simulink model "dc_voltage_control_A"  (R2018b)
settings: Solver=ode45  StartTime=0.0  StopTime=90  MaxStep=100e-6  RelTol=1e-3
PreLoadFcn:
  | load_system('../simulink_reference_models/test_sequence_lib');
InitFcn:
  | close all
  | clear all
  | 
  | T_CNTL = 1/5e3;
  | 
  | VLL_NOM = 480;
  | F_NOM = 60;
  | VLL_INV_NOM = VLL_NOM;
  | S_RATED = 1e6;
  | I_BASE = S_RATED / (sqrt(3) * VLL_NOM);
  | 
  | V_LVDC_NOM = 0.0; % to make cap voltage start from 0
  | C_DC = 50e-3;
libraries: simulink x12, test_sequence_lib x6, controls_element_lib x1
settings Model: SimulationMode=accelerator  Creator=HussamAlatrash  LastModifiedBy=ahhei
settings DataIOCC: ReturnWorkspaceOutputs=on
settings DebuggingCC: UnconnectedInputMsg=none  UnconnectedOutputMsg=none  UnconnectedLineMsg=none
settings ModelReferenceCC: EnableRefExpFcnMdlSchedulingChecks=off
settings RTWCC: Description=Generic Real-Time Target
settings ConfigComp: CovBoundaryAbsTol=1.0e-5

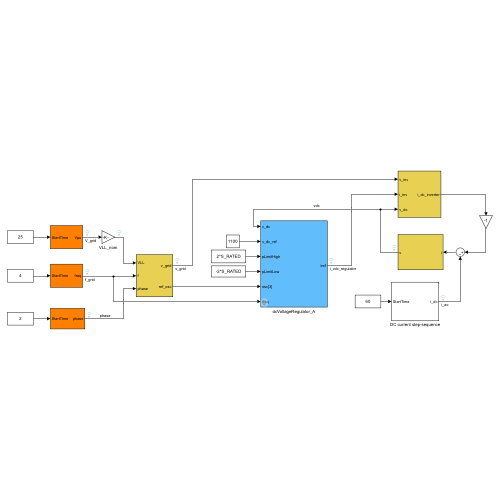
[thumbnail: Simulink's stored preview of the top-level diagram]
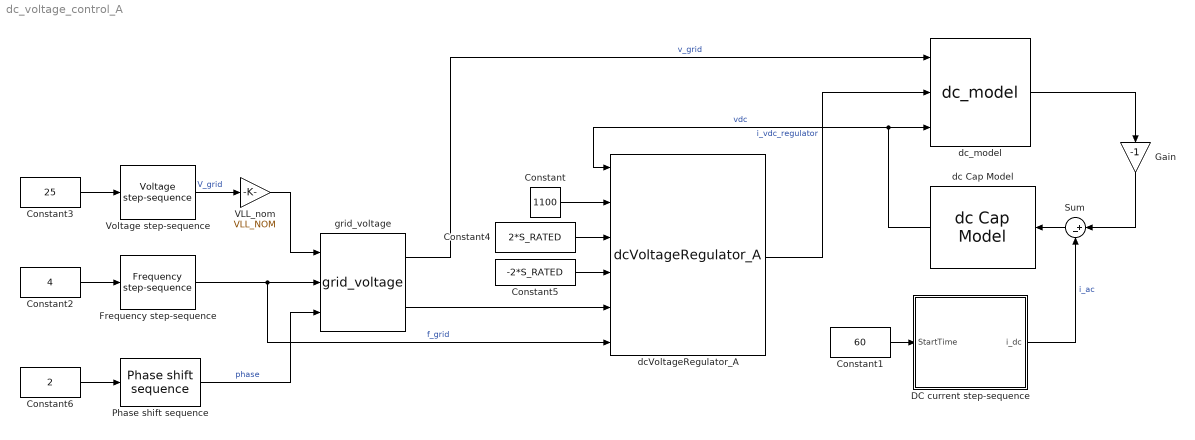
== system dc_voltage_control_A ==
  Constant : Constant  Value=1100
  Constant1 : Constant  Value=60
  Constant2 : Constant  Value=4
  Constant3 : Constant  Value=25
  Constant4 : Constant  Value=2*S_RATED
  Constant5 : Constant  Value=-2*S_RATED
  Constant6 : Constant  Value=2
  DC current step-sequence : Subsystem
  Frequency step-sequence : test_sequence_lib/Frequency step-sequence  SystemSampleTime=-1  EmptyChoice=off  PassThrough=off  PassThroughVariantControl=(default)  EmptyChoiceVariantControl=(default)  Latency=0  AutoFrameSizeCalculation=off
  Gain : Gain  Gain=-1
  Phase shift sequence : test_sequence_lib/Phase shift sequence  SystemSampleTime=-1  EmptyChoice=off  PassThrough=off  PassThroughVariantControl=(default)  EmptyChoiceVariantControl=(default)  Latency=0  AutoFrameSizeCalculation=off
  Sum : Sum  Inputs=|+-
  VLL_nom : Gain  Gain=VLL_NOM
  Voltage step-sequence : test_sequence_lib/Voltage step-sequence  SystemSampleTime=-1  EmptyChoice=off  PassThrough=off  PassThroughVariantControl=(default)  EmptyChoiceVariantControl=(default)  Latency=0  AutoFrameSizeCalculation=off
  dc Cap Model : test_sequence_lib/dc Cap Model  SystemSampleTime=-1  EmptyChoice=off  PassThrough=off  PassThroughVariantControl=(default)  EmptyChoiceVariantControl=(default)  Latency=0  AutoFrameSizeCalculation=off
  dcVoltageRegulator_A : controls_element_lib/dcVoltageRegulator_A  kp=20e3  kSlowPath=0  wSlowPath=5  pLimitExternalMinimum=0  vdc_deadband=0  VllRated=VLL_INV_NOM
  dc_model : test_sequence_lib/dc_model  SystemSampleTime=-1  EmptyChoice=off  PassThrough=off  PassThroughVariantControl=(default)  EmptyChoiceVariantControl=(default)  Latency=0  AutoFrameSizeCalculation=off
  grid_voltage : test_sequence_lib/grid_voltage  SystemSampleTime=-1  EmptyChoice=off  PassThrough=off  PassThroughVariantControl=(default)  EmptyChoiceVariantControl=(default)  Latency=0  AutoFrameSizeCalculation=off
  wires:
  Constant2/1 -> Frequency step-sequence/1
  Constant3/1 -> Voltage step-sequence/1
  Constant6/1 -> Phase shift sequence/1
  VLL_nom/1 -> grid_voltage/1
  Voltage step-sequence/1 -> VLL_nom/1  "V_grid"
  Frequency step-sequence/1 -> dcVoltageRegulator_A/6, grid_voltage/2  "f_grid"
  Phase shift sequence/1 -> grid_voltage/3  "phase"
  Constant5/1 -> dcVoltageRegulator_A/4
  Constant4/1 -> dcVoltageRegulator_A/3
  dcVoltageRegulator_A/1 -> dc_model/2  "i_vdc_regulator"
  grid_voltage/2 -> dcVoltageRegulator_A/5
  grid_voltage/1 -> dc_model/1  "v_grid"
  dc_model/1 -> Gain/1
  dc Cap Model/1 -> dc_model/3, dcVoltageRegulator_A/1  "vdc"
  Constant/1 -> dcVoltageRegulator_A/2
  Gain/1 -> Sum/1
  Constant1/1 -> DC current step-sequence/1(StartTime)
  Sum/1 -> dc Cap Model/1
  DC current step-sequence/1(i_dc) -> Sum/2  "i_ac"

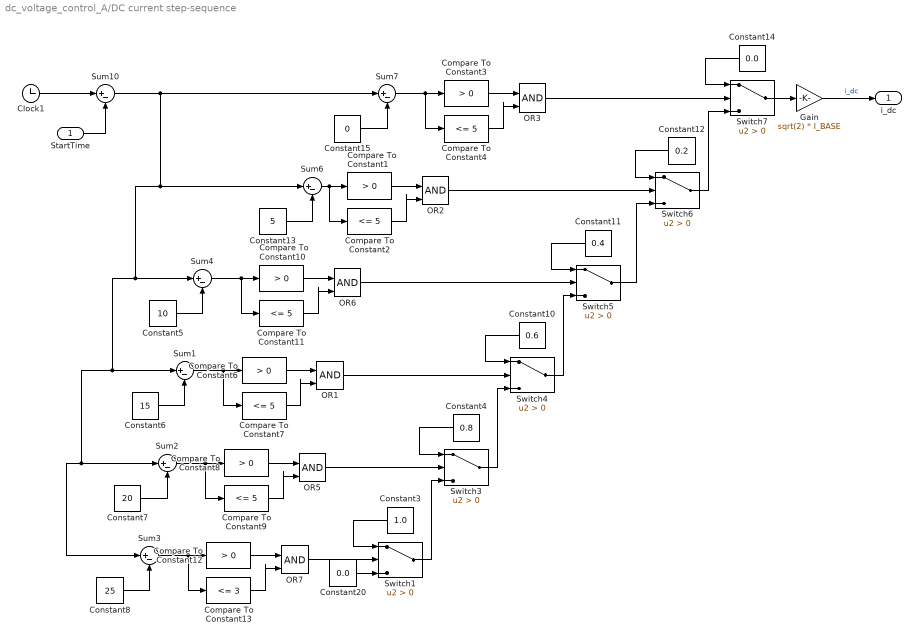
== system dc_voltage_control_A/DC current step-sequence ==
  StartTime : Inport
  Clock1 : Clock
  Compare To Constant{1,3,6,8,10,12} (6 alike) : simulink/Logic and Bit Operations/Compare To Constant  relop=>  const=0  OutDataTypeStr=boolean
  Compare To Constant{2,4,7,9,11} (5 alike) : simulink/Logic and Bit Operations/Compare To Constant  relop=<=  const=5  OutDataTypeStr=boolean
  Compare To Constant13 : simulink/Logic and Bit Operations/Compare To Constant  relop=<=  const=3  OutDataTypeStr=boolean
  Constant10 : Constant  Value=0.6
  Constant11 : Constant  Value=0.4
  Constant12 : Constant  Value=0.2
  Constant13 : Constant  Value=5
  Constant14 : Constant  Value=0.0
  Constant15 : Constant  Value=0
  Constant20 : Constant  Value=0.0
  Constant3 : Constant  Value=1.0
  Constant4 : Constant  Value=0.8
  Constant5 : Constant  Value=10
  Constant6 : Constant  Value=15
  Constant7 : Constant  Value=20
  Constant8 : Constant  Value=25
  Gain : Gain  Gain=sqrt(2) * I_BASE
  OR{1..3,5..7} (6 alike) : Logic  IconShape=distinctive  AllPortsSameDT=off  OutDataTypeStr=boolean
  Sum{1..4,6..7,10} (7 alike) : Sum  Inputs=|+-
  Switch{1,3..7} (6 alike) : Switch  Criteria=u2 > Threshold
  i_dc : Outport
  wires:
  StartTime/1 -> Sum10/2
  Clock1/1 -> Sum10/1
  Sum7/1 -> Compare To Constant4/1, Compare To Constant3/1
  Constant11/1 -> Switch5/1
  Compare To Constant4/1 -> OR3/2
  Compare To Constant6/1 -> OR1/1
  Sum10/1 -> Sum7/1, Sum2/1, Sum3/1, Sum1/1, Sum4/1, Sum6/1
  Constant7/1 -> Sum2/2
  Constant10/1 -> Switch4/1
  Compare To Constant1/1 -> OR2/1
  Compare To Constant10/1 -> OR6/1
  Compare To Constant12/1 -> OR7/1
  Switch5/1 -> Switch6/3
  OR7/1 -> Switch1/2
  Sum6/1 -> Compare To Constant1/1, Compare To Constant2/1
  Constant6/1 -> Sum1/2
  Compare To Constant8/1 -> OR5/1
  Sum1/1 -> Compare To Constant6/1, Compare To Constant7/1
  Constant14/1 -> Switch7/1
  Constant13/1 -> Sum6/2
  Gain/1 -> i_dc/1  "i_dc"
  Switch6/1 -> Switch7/3
  Constant12/1 -> Switch6/1
  Compare To Constant9/1 -> OR5/2
  Sum2/1 -> Compare To Constant9/1, Compare To Constant8/1
  Constant4/1 -> Switch3/1
  Constant8/1 -> Sum3/2
  Switch3/1 -> Switch4/3
  Constant5/1 -> Sum4/2
  OR1/1 -> Switch4/2
  Constant20/1 -> Switch1/3
  Compare To Constant2/1 -> OR2/2
  Sum3/1 -> Compare To Constant12/1, Compare To Constant13/1
  Compare To Constant3/1 -> OR3/1
  OR2/1 -> Switch6/2
  Compare To Constant7/1 -> OR1/2
  Switch1/1 -> Switch3/3
  Compare To Constant11/1 -> OR6/2
  OR5/1 -> Switch3/2
  Sum4/1 -> Compare To Constant11/1, Compare To Constant10/1
  Constant3/1 -> Switch1/1
  Switch4/1 -> Switch5/3
  OR6/1 -> Switch5/2
  Switch7/1 -> Gain/1
  Compare To Constant13/1 -> OR7/2
  OR3/1 -> Switch7/2
  Constant15/1 -> Sum7/2
